simulink model "ContBas"  (R2026b)
settings: Solver=FixedStepAuto  StopTime=inf  EnableMultiTasking=on
libraries: px4uORBlib x2, px4Peripheralslib x1
settings Model: Creator=cfmm  LastModifiedBy=cfmm
settings SolverCC: PositivePriorityOrder=on
settings OptimizationCC: DifferentSizesBufferReuse=on  EfficientTunableParamExpr=on  EnhancedBackFolding=on  MaxStackSize=64  OptimizationCustomize=off  OptimizeBlockOrder=speed  PassReuseOutputArgsAs=Individual arguments  RemoveInternalMemoryZeroInit=on  RemoveRootLevelIOMemoryZeroInit=on
settings DebuggingCC: ParameterTunabilityLossMsg=error
settings HardwareCC: ProdHWDeviceType=ARM Compatible->ARM Cortex  ProdLargestAtomicFloat=Double  ProdLargestAtomicInteger=Long  ProdLongLongMode=on
settings SFSimCC: MATLABDynamicMemAlloc=off  SimTargetLang=C++
settings RTWCC: Description=Embedded Coder  HardwareBoard=PX4 Host Target  PortableWordSizes=on  SystemTargetFile=ert.tlc  TLCOptions="-aInlineSetEventsForThisBaseRateFcn=TLC_FALSE -aSuppressMultiTaskScheduler=TLC_FALSE  -aRateBasedStepFcn=0"  TargetLang=C++  TemplateMakefile=ert_default_tmf  Toolchain=GNU Tools for PX4 Autopilots
settings CodeAppCC: ForceParamTrailComments=on  IgnoreCustomStorageClasses=off  InsertBlockDesc=on  OperatorAnnotations=on  SFDataObjDesc=on  SimulinkDataObjDesc=on
settings ERTTargetCC: CombineSignalStateStructs=on  ExtModeIntrfLevel=Level2 - Open  ExtModeMexFile=ext_xcp  ExtModeStaticAlloc=on

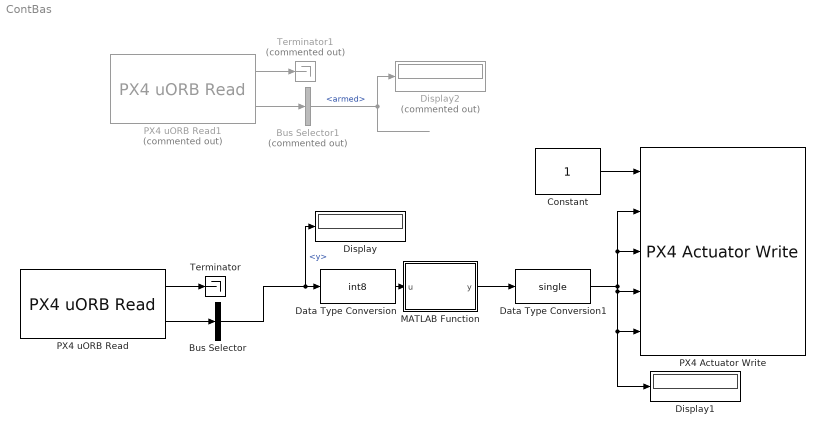
== system ContBas ==
  Bus Selector : BusSelector  OutputSignals=y
  Bus Selector1 : BusSelector  Commented=on  OutputSignals=armed
  Constant : Constant  OutDataTypeStr=boolean
  Data Type Conversion : DataTypeConversion  OutDataTypeStr=int8  SaturateOnIntegerOverflow=off  RndMeth=Floor
  Data Type Conversion1 : DataTypeConversion  OutDataTypeStr=single  SaturateOnIntegerOverflow=off  RndMeth=Floor
  Display : Display
  Display1 : Display
  Display2 : Display  Commented=on
  MATLAB Function : MATLAB Function  TreatAsAtomicUnit=on
  PX4 Actuator Write : px4Peripheralslib/PX4 Actuator Write  Motor1Enable=on  Motor2Enable=on  Motor3Enable=on  Motor4Enable=on  Motor5Enable=off  Motor6Enable=off  Motor7Enable=off  Motor8Enable=off  Motor9Enable=off  Motor10Enable=off  Motor11Enable=off  Motor12Enable=off  IsMotorArray=off  Servo1Enable=off  Servo2Enable=off  Servo3Enable=off  Servo4Enable=off  Servo5Enable=off  Servo6Enable=off  Servo7Enable=off  Servo8Enable=off  IsServoArray=off
  PX4 uORB Read : px4uORBlib/PX4 uORB Read  uORBMsg=SensorGyro  uORBTopicName=sensor_gyro  SubscribeNonZeroInstance=off  selectInstanceNum=1  SampleTime=0.01  isSingleTopicMsg=on  BlockingMode=off  BlockTimeout=1e-3
  PX4 uORB Read1 : px4uORBlib/PX4 uORB Read  Commented=on  uORBMsg=ActuatorArmed  uORBTopicName=actuator_armed  SubscribeNonZeroInstance=off  selectInstanceNum=1  SampleTime=0.01  isSingleTopicMsg=on  BlockingMode=off  BlockTimeout=1e-3
  Terminator : Terminator
  Terminator1 : Terminator  Commented=on
  wires:
  Bus Selector1/1 -> Display2/1  "<armed>"
  MATLAB Function/1(y) -> Data Type Conversion1/1
  PX4 uORB Read/2 -> Bus Selector/1
  Bus Selector/1 -> Data Type Conversion/1, Display/1  "<y>"
  Data Type Conversion/1 -> MATLAB Function/1(u)
  Data Type Conversion1/1 -> PX4 Actuator Write/4, PX4 Actuator Write/5, Display1/1, PX4 Actuator Write/3, PX4 Actuator Write/2
  PX4 uORB Read/1 -> Terminator/1
  PX4 uORB Read1/1 -> Terminator1/1
  PX4 uORB Read1/2 -> Bus Selector1/1
  Constant/1 -> PX4 Actuator Write/1

== matlab function ContBas/MATLAB Function ==
  data: u input; y output
function y = fcn(u)
if (u > 5)
    y = 0.1;
else
    y = 0.7;
end
